simulink model "Assembly_Upperstage"  (R2023b)
settings: Solver=VariableStepAuto  StartTime=0.0  StopTime=30  RelTol=1e-3
InitFcn:
  | addpath(pwd);
  | run('Assembly_Upperstage_DataFile.m');
  | disp('✅ InitFcn executed: Path added and data file loaded.');
model workspace: external: MAT-File C:\Program Files\MATLAB\R2023b\bin\win64\Assembly_Upperstage_DataFile1.mat (data not in the file)
undefined symbols (not defined in the file or in its folder): smiData, X, Y, Z
libraries: sm_lib x49, nesl_utility x4
(part 2 of 2)

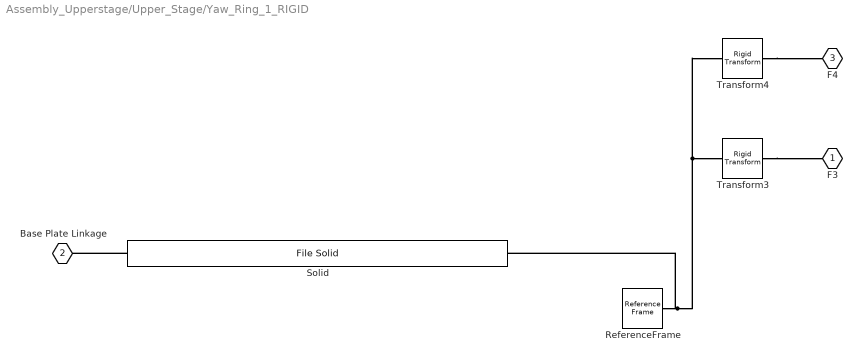
== system Assembly_Upperstage/Upper_Stage/Yaw_Ring_1_RIGID ==
  ReferenceFrame : sm_lib/Frames and Transforms/Reference Frame
  Solid : sm_lib/Body Elements/File Solid  ExtGeomFileName=Yaw_Ring_Default_sldprt.STEP  UnitType=FromFile  ExtGeomFileUnits=m  StepReaderType=HEX  ExportConvexHullGeometry=off  InertiaType=Custom  Mass=smiData.Solid(6).mass  MassUnits=kg  CenterOfMass=smiData.Solid(6).CoM  CenterOfMassUnits=mm  MomentsOfInertia=smiData.Solid(6).MoI  MomentsOfInertiaUnits=kg*mm^2  ProductsOfInertia=smiData.Solid(6).PoI  ProductsOfInertiaUnits=kg*mm^2  BasedOnType=DensityFromFile  Density=1000  DensityUnits=kg/m^3  DoExposeReferenceFrame=on  SerializedFrames=<Frames><Frame><Id>Frame1</Id><Value><Name>Base PLate Linkage</Name><Origin><Source>GeometricFeature</Source><FeatureName>circular curve 4</FeatureName></Origin><PrimaryAxis><DefinedDirection>+Z</DefinedDirection><Source>GeometricFeature</Source><SourceDirection>+Z</SourceDirection><FeatureName>planar surface 3</FeatureName></PrimaryAxis><SecondaryAxis><DefinedDirection>+X</DefinedDirection><Source>GeometricFeature</Source><SourceDirection>+X</SourceDirection><FeatureName>planar surface 28</FeatureName></SecondaryAxis></Value></Frame></Frames>  GraphicType=FromGeometry  MarkerShape=Sphere  MarkerSize=10  GraphicVisPropType=SimpleVisualProperties  GraphicDiffuseColor=smiData.Solid(6).color  GraphicSpecularColor=[0.5 0.5 0.5 1.0]  GraphicAmbientColor=[0.15 0.15 0.15 1.0]  GraphicEmissiveColor=[0.0 0.0 0.0 1.0]  GraphicShininess=75  GraphicOpacity=smiData.Solid(6).opacity
  Transform3 : sm_lib/Frames and Transforms/Rigid Transform  TranslationMethod=Cartesian  TranslationStandardOffset=0  TranslationStandardOffsetUnits=m  TranslationStandardAxis=+Z  TranslationCartesianOffset=smiData.RigidTransform(23).translation  TranslationCartesianOffsetUnits=mm  TranslationROffset=0  TranslationROffsetUnits=m  TranslationZOffset=0  TranslationZOffsetUnits=m  TranslationThetaOffset=0  TranslationThetaOffsetUnits=deg  RotationMethod=ArbitraryAxis  RotationAngleUnits=rad  RotationStandardAxis=+Z  RotationAngle=smiData.RigidTransform(23).angle  RotationArbitraryAxis=smiData.RigidTransform(23).axis  FollAlignAxisA=+X  BaseAlignAxisA=+Y  FollAlignAxisB=+Y  BaseAlignAxisB=+Z  RotationSequenceAxes=FollowerAxes  RotationSequence=XYX  RotationSequenceAngles=[0 0 0]  RotationSequenceAnglesUnits=deg  RotationMatrix=[1 0 0; 0 1 0; 0 0 1]  Quaternion=[1 0 0 0]
  Transform4 : sm_lib/Frames and Transforms/Rigid Transform  TranslationMethod=Cartesian  TranslationStandardOffset=0  TranslationStandardOffsetUnits=m  TranslationStandardAxis=+Z  TranslationCartesianOffset=smiData.RigidTransform(25).translation  TranslationCartesianOffsetUnits=mm  TranslationROffset=0  TranslationROffsetUnits=m  TranslationZOffset=0  TranslationZOffsetUnits=m  TranslationThetaOffset=0  TranslationThetaOffsetUnits=deg  RotationMethod=ArbitraryAxis  RotationAngleUnits=rad  RotationStandardAxis=+Z  RotationAngle=smiData.RigidTransform(25).angle  RotationArbitraryAxis=smiData.RigidTransform(25).axis  FollAlignAxisA=+X  BaseAlignAxisA=+Y  FollAlignAxisB=+Y  BaseAlignAxisB=+Z  RotationSequenceAxes=FollowerAxes  RotationSequence=XYX  RotationSequenceAngles=[0 0 0]  RotationSequenceAnglesUnits=deg  RotationMatrix=[1 0 0; 0 1 0; 0 0 1]  Quaternion=[1 0 0 0]
  F3 : PMIOPort  Side=Left
  Base Plate Linkage : PMIOPort  Port=2  Side=Right
  F4 : PMIOPort  Port=3  Side=Right
  connections:
  Solid/RConn1 -- Transform3/LConn1 -- Transform4/LConn1 -- ReferenceFrame/RConn1
  Transform3/RConn1 -- F3/RConn1
  Transform4/RConn1 -- F4/RConn1
  Solid/LConn1 -- Base Plate Linkage/RConn1

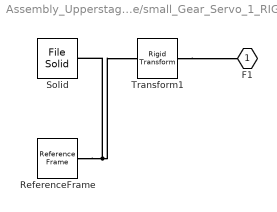
== system Assembly_Upperstage/Upper_Stage/small_Gear_Servo_1_RIGID ==
  ReferenceFrame : sm_lib/Frames and Transforms/Reference Frame
  Solid : sm_lib/Body Elements/File Solid  ExtGeomFileName=small Gear_Servo__Default_sldprt.STEP  UnitType=FromFile  ExtGeomFileUnits=m  StepReaderType=HEX  ExportConvexHullGeometry=off  InertiaType=Custom  Mass=smiData.Solid(13).mass  MassUnits=kg  CenterOfMass=smiData.Solid(13).CoM  CenterOfMassUnits=mm  MomentsOfInertia=smiData.Solid(13).MoI  MomentsOfInertiaUnits=kg*mm^2  ProductsOfInertia=smiData.Solid(13).PoI  ProductsOfInertiaUnits=kg*mm^2  BasedOnType=DensityFromFile  Density=1000  DensityUnits=kg/m^3  DoExposeReferenceFrame=on  SerializedFrames=<Frames/>  GraphicType=FromGeometry  MarkerShape=Sphere  MarkerSize=10  GraphicVisPropType=SimpleVisualProperties  GraphicDiffuseColor=smiData.Solid(13).color  GraphicSpecularColor=[0.5 0.5 0.5 1.0]  GraphicAmbientColor=[0.15 0.15 0.15 1.0]  GraphicEmissiveColor=[0.0 0.0 0.0 1.0]  GraphicShininess=75  GraphicOpacity=smiData.Solid(13).opacity
  Transform1 : sm_lib/Frames and Transforms/Rigid Transform  TranslationMethod=Cartesian  TranslationStandardOffset=0  TranslationStandardOffsetUnits=m  TranslationStandardAxis=+Z  TranslationCartesianOffset=smiData.RigidTransform(37).translation  TranslationCartesianOffsetUnits=mm  TranslationROffset=0  TranslationROffsetUnits=m  TranslationZOffset=0  TranslationZOffsetUnits=m  TranslationThetaOffset=0  TranslationThetaOffsetUnits=deg  RotationMethod=ArbitraryAxis  RotationAngleUnits=rad  RotationStandardAxis=+Z  RotationAngle=smiData.RigidTransform(37).angle  RotationArbitraryAxis=smiData.RigidTransform(37).axis  FollAlignAxisA=+X  BaseAlignAxisA=+Y  FollAlignAxisB=+Y  BaseAlignAxisB=+Z  RotationSequenceAxes=FollowerAxes  RotationSequence=XYX  RotationSequenceAngles=[0 0 0]  RotationSequenceAnglesUnits=deg  RotationMatrix=[1 0 0; 0 1 0; 0 0 1]  Quaternion=[1 0 0 0]
  F1 : PMIOPort  Side=Right
  connections:
  Solid/RConn1 -- ReferenceFrame/RConn1 -- Transform1/LConn1
  Transform1/RConn1 -- F1/RConn1

== matlab function Assembly_Upperstage/Upper_Stage/MATLAB Function ==
  data: t input; y output
function y = fcn(t)
  A = deg2rad(30);  % 30° in radians
  f = 0.3;            % Frequency in Hz
  y = A * sin(2*pi*f*t);
end

== matlab function Assembly_Upperstage/Upper_Stage/MATLAB Function2 ==
  data: t input; y output
function y = fcn(t)
  A = deg2rad(30);  % 30° in radians
  f = 0.3;            % Frequency in Hz
  y = A * sin(2*pi*f*t);
end

== matlab function Assembly_Upperstage/Upper_Stage/MATLAB Function1 ==
  data: t input; y output
function y = fcn(t)
  A = deg2rad(30);  % 30° in radians
  f = 0.3;            % Frequency in Hz
  y = A * sin(2*pi*f*t)+pi/2;
end
